simulink model "soc_03_1rc_ekf"  (R2025a)
settings: Solver=FixedStepDiscrete  StartTime=0.0  StopTime=240  FixedStep=dt  RelTol=1e-3
model workspace (MAT data in the model file):
  R0 = 0.05
  R1 = 0.03
  capacityAh = 2
  dt = 1
  ocvCubic = 0.6
  ocvLinear = 0.006
  ocvOffset = 3
  tau1 = 20
  voltageVariance = 0.0004
undefined symbols (not defined in the file): DiscIntNeverNeededParam
Description:
  | Lesson 3: 1RC battery model and EKF with a synthetic OCV curve. Use Compare SOC and Terminal voltage. After discharge stops at t=60 s, SOC stays constant while the RC polarization voltage decays. Cell values are stored in Model Workspace; they are illustrative, not fitted to a real cell.
settings Model: Creator=mosri  LastModifiedBy=mosri

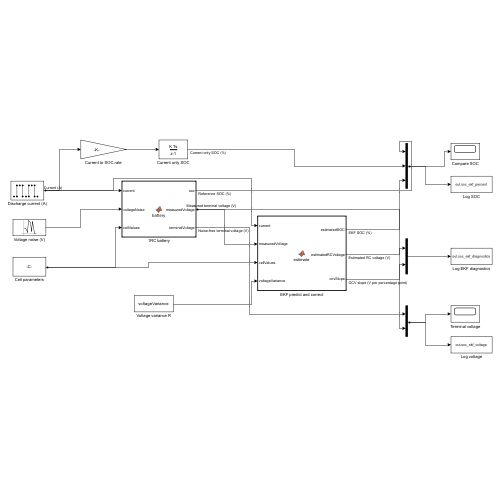
[thumbnail: Simulink's stored preview of the top-level diagram]
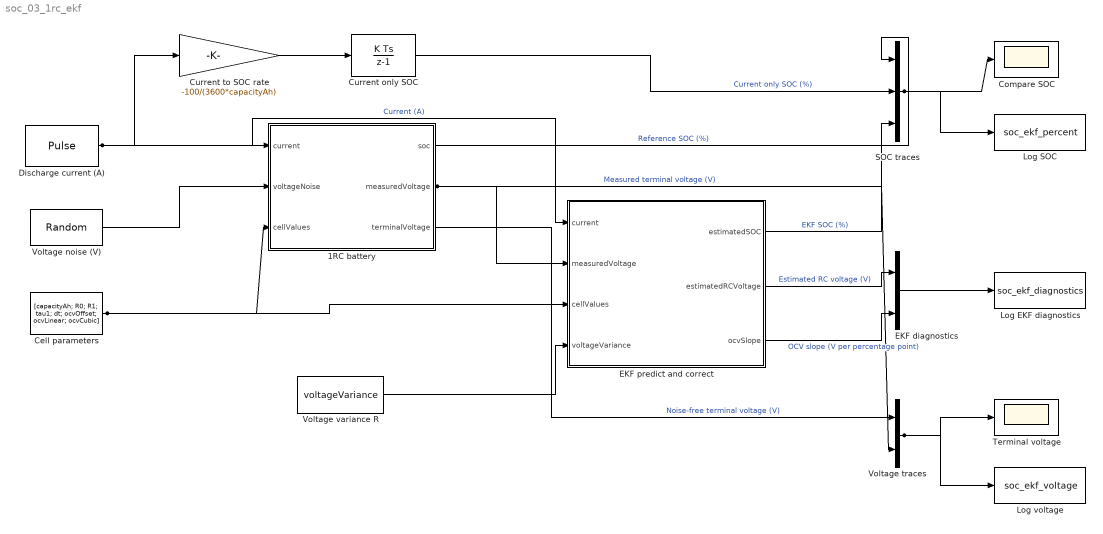
== system soc_03_1rc_ekf ==
  1RC battery : MATLAB Function  TreatAsAtomicUnit=on
  Cell parameters : Constant  Value=[capacityAh; R0; R1; tau1; dt; ocvOffset; ocvLinear; ocvCubic]  SampleTime=dt
  Compare SOC : Scope
      settings: Title=Reference, current only, and EKF  ActiveDisplayYMinimum=45  ActiveDisplayYMaximum=85  YLabel=SOC (%)
  Current only SOC : DiscreteIntegrator  InitialCondition=50  SampleTime=dt  ICPrevOutput=DiscIntNeverNeededParam  ICPrevScaledInput=DiscIntNeverNeededParam
  Current to SOC rate : Gain  Gain=-100/(3600*capacityAh)
  Discharge current (A) : DiscretePulseGenerator  Period=120  PulseWidth=60  SampleTime=dt
  EKF diagnostics : Mux  Inputs=2
  EKF predict and correct : MATLAB Function  TreatAsAtomicUnit=on
  Log EKF diagnostics : ToWorkspace  VariableName=soc_ekf_diagnostics  SampleTime=-1
  Log SOC : ToWorkspace  VariableName=soc_ekf_percent  SampleTime=-1
  Log voltage : ToWorkspace  VariableName=soc_ekf_voltage  SampleTime=-1
  SOC traces : Mux  Inputs=3
  Terminal voltage : Scope
      settings: Title=Terminal voltage during discharge and rest  ActiveDisplayYMinimum=3.55  ActiveDisplayYMaximum=3.9  YLabel=Terminal voltage (V)
  Voltage noise (V) : RandomNumber  Variance=voltageVariance  Seed=42  SampleTime=dt
  Voltage traces : Mux  Inputs=2
  Voltage variance R : Constant  Value=voltageVariance  SampleTime=dt
  wires:
  Discharge current (A)/1 -> Current to SOC rate/1, 1RC battery/1(current), EKF predict and correct/1(current)  "Current (A)"
  Current to SOC rate/1 -> Current only SOC/1
  Current only SOC/1 -> SOC traces/2  "Current only SOC (%)"
  Voltage noise (V)/1 -> 1RC battery/2(voltageNoise)
  Cell parameters/1 -> 1RC battery/3(cellValues), EKF predict and correct/3(cellValues)
  1RC battery/1(soc) -> SOC traces/1  "Reference SOC (%)"
  1RC battery/2(measuredVoltage) -> EKF predict and correct/2(measuredVoltage), Voltage traces/2  "Measured terminal voltage (V)"
  1RC battery/3(terminalVoltage) -> Voltage traces/1  "Noise-free terminal voltage (V)"
  Voltage variance R/1 -> EKF predict and correct/4(voltageVariance)
  EKF predict and correct/1(estimatedSOC) -> SOC traces/3  "EKF SOC (%)"
  EKF predict and correct/2(estimatedRCVoltage) -> EKF diagnostics/1  "Estimated RC voltage (V)"
  EKF predict and correct/3(ocvSlope) -> EKF diagnostics/2  "OCV slope (V per percentage point)"
  SOC traces/1 -> Compare SOC/1, Log SOC/1
  Voltage traces/1 -> Terminal voltage/1, Log voltage/1
  EKF diagnostics/1 -> Log EKF diagnostics/1

== matlab function soc_03_1rc_ekf/EKF predict and correct ==
  data: current input; estimatedSOC output; measuredVoltage input; cellValues input; voltageVariance input; estimatedRCVoltage output; ocvSlope output
function [estimatedSOC, estimatedRCVoltage, ocvSlope] = estimate(current, measuredVoltage, cellValues, voltageVariance)
% x = [SOC in percent; RC polarization voltage in volts].
persistent x P previousCurrent
if isempty(x)
    x = [50; 0];
    P = diag([10^2, 0.01^2]);      % Initial uncertainty (SOC and RC voltage)
    previousCurrent = current;
else
    % 1. Predict both states using current from the previous interval.
    dt = cellValues(5);
    a = exp(-dt/cellValues(4));
    A = [1 0; 0 a];
    B = [-100*dt/(3600*cellValues(1)); (1-a)*cellValues(3)];
    Q = diag([1e-3, 1e-6]);        % Per-sample process noise variances
    xPred = A*x + B*previousCurrent;
    PPred = A*P*A' + Q;

    % 2. Predict terminal voltage using the nonlinear OCV curve.
    soc = xPred(1);
    ocv = cellValues(6) + cellValues(7)*soc + cellValues(8)*(soc/100)^3;
    predictedVoltage = ocv - cellValues(2)*current - xPred(2);

    % 3. Linearize the observation at the predicted SOC, then correct.
    ocvSlope = cellValues(7) + 3*cellValues(8)*(soc/100)^2/100;
    H = [ocvSlope, -1];
    innovation = measuredVoltage - predictedVoltage;
    K = (PPred*H')/(H*PPred*H' + voltageVariance);
    x = xPred + K*innovation;

    % Joseph form keeps the covariance symmetric and nonnegative.
    M = eye(2) - K*H;
    P = M*PPred*M' + K*voltageVariance*K';
    previousCurrent = current;
    estimatedSOC = x(1);
    estimatedRCVoltage = x(2);
    return
end
estimatedSOC = x(1);
estimatedRCVoltage = x(2);
ocvSlope = cellValues(7) + 3*cellValues(8)*(x(1)/100)^2/100;
end

== matlab function soc_03_1rc_ekf/1RC battery ==
  data: current input; soc output; voltageNoise input; cellValues input; measuredVoltage output; terminalVoltage output
function [soc, measuredVoltage, terminalVoltage] = battery(current, voltageNoise, cellValues)
% Positive current discharges the cell. SOC uses 0 to 100 percent.
% cellValues = [capacityAh; R0; R1; tau1; dt; ocvOffset; ocvLinear; ocvCubic].
persistent charge polarization previousCurrent
if isempty(charge)
    charge = 80;
    polarization = 0;
    previousCurrent = current;
else
    dt = cellValues(5);
    a = exp(-dt/cellValues(4));
    charge = charge - 100*dt*previousCurrent/(3600*cellValues(1));
    polarization = a*polarization + (1-a)*cellValues(3)*previousCurrent;
    previousCurrent = current;
end

soc = charge;
ocv = cellValues(6) + cellValues(7)*soc + cellValues(8)*(soc/100)^3;
terminalVoltage = ocv - cellValues(2)*current - polarization;
measuredVoltage = terminalVoltage + voltageNoise;
end
